simulink model "endocrino"  (R2026b)
settings: Solver=ode15s  StopTime=10  MaxStep=1E-3
libraries: slpidlib x1
settings Model: Creator=BioMath  LastModifiedBy=Emiliano
settings DataIOCC: DSMLogging=off  ReturnWorkspaceOutputs=off  SaveOutput=off  SignalLogging=off  TimeSaveName=t
settings DebuggingCC: AlgebraicLoopMsg=none  ArtificialAlgebraicLoopMsg=none  MaxConsecutiveZCsMsg=none

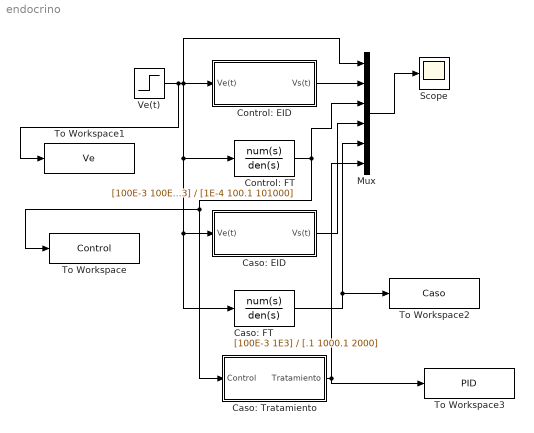
== system endocrino ==
  Caso: EID : Subsystem
  Caso: FT : TransferFcn  Numerator=[100E-3 1E3]  Denominator=[.1 1000.1 2000]
  Caso: Tratamiento : Subsystem
  Control: EID : Subsystem
  Control: FT : TransferFcn  Numerator=[100E-3 100E3]  Denominator=[1E-4 100.1 101000]
  Mux : Mux  Inputs=6
  Scope : Scope
      settings: ActiveDisplayYMinimum=0  ActiveDisplayYMaximum=1.1
  To Workspace : ToWorkspace  VariableName=Control  SampleTime=-1
  To Workspace1 : ToWorkspace  VariableName=Ve  SampleTime=-1
  To Workspace2 : ToWorkspace  VariableName=Caso  SampleTime=-1
  To Workspace3 : ToWorkspace  VariableName=PID  SampleTime=-1
  Ve(t) : Step  Time=0  SampleTime=0
  wires:
  Ve(t)/1 -> To Workspace1/1, Caso: FT/1, Caso: EID/1(Ve(t)), Control: FT/1, Control: EID/1(Ve(t)), Mux/1
  Control: EID/1(Vs(t)) -> Mux/2
  Mux/1 -> Scope/1
  Control: FT/1 -> To Workspace/1, Caso: Tratamiento/1(Control), Mux/3
  Caso: EID/1(Vs(t)) -> Mux/4
  Caso: FT/1 -> To Workspace2/1, Mux/5
  Caso: Tratamiento/1(Tratamiento) -> Mux/6, To Workspace3/1

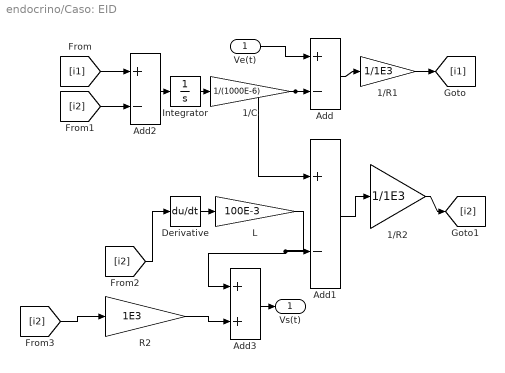
== system endocrino/Caso: EID ==
  Ve(t) : Inport
  1/C : Gain  Gain=1/(1000E-6)
  1/R1 : Gain  Gain=1/1E3
  1/R2 : Gain  Gain=1/1E3
  Add : Sum  Inputs=+-
  Add1 : Sum  Inputs=+-
  Add2 : Sum  Inputs=+-
  Add3 : Sum
  Derivative : Derivative
  Integrator : Integrator
  L : Gain  Gain=100E-3
  R2 : Gain  Gain=1E3
  Vs(t) : Outport
  wires:
  Add1/1 -> 1/R2/1
  1/R2/1 -> [i2]
  Derivative/1 -> L/1
  L/1 -> Add3/1, Add1/2
  1/R1/1 -> [i1]
  Add/1 -> 1/R1/1
  Ve(t)/1 -> Add/1
  [i2] -> Add2/2
  [i1] -> Add2/1
  Add2/1 -> Integrator/1
  Integrator/1 -> 1/C/1
  1/C/1 -> Add1/1, Add/2
  [i2] -> Derivative/1
  [i2] -> R2/1
  R2/1 -> Add3/2
  Add3/1 -> Vs(t)/1

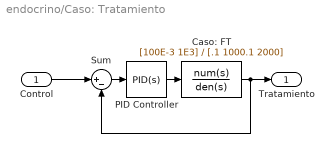
== system endocrino/Caso: Tratamiento ==
  Control : Inport
  Caso: FT : TransferFcn  Numerator=[100E-3 1E3]  Denominator=[.1 1000.1 2000]
  PID Controller : slpidlib/PID Controller  Controller=PID  Form=Parallel  TimeDomain=Continuous-time  UseExternalTs=off  SampleTime=-1  IntegratorMethod=Forward Euler  FilterMethod=Forward Euler  ControllerParametersSource=internal  P=529.0879  I=51836.0493  UseKiTs=off  D=0.17756  UseExternalDerivativeSource=off  N=2021.2211  UseFilter=on  TunerSelectOption=Transfer Function Based (PID Tuner App)  InitialConditionSource=internal  InitialConditionForIntegrator=0  InitialConditionForFilter=0  DifferentiatorICPrevScaledInput=0  ExternalReset=none  TrackingMode=off  Kt=1  LimitOutput=off  SatLimitsSource=internal  UpperSaturationLimit=inf  LowerSaturationLimit=-inf  LinearizeAsGain=on  AntiWindupMode=none  Kb=1  LimitIntegrator=off  UpperIntegratorSaturationLimit=inf  LowerIntegratorSaturationLimit=-inf  POutMin=[]  POutMax=[]  IOutMin=[]  IOutMax=[]  DOutMin=[]  DOutMax=[]  NOutMin=[]  NOutMax=[]  SumOutMin=[]  SumOutMax=[]  SaturationOutMin=[]  SaturationOutMax=[]  PParamMin=[]  PParamMax=[]  IParamMin=[]  IParamMax=[]  DParamMin=[]  DParamMax=[]  NParamMin=[]  NParamMax=[]  KbParamMin=[]  KbParamMax=[]  KtParamMin=[]  KtParamMax=[]  KbOutMin=[]  KbOutMax=[]  KtOutMin=[]  KtOutMax=[]  IntegratorOutMin=[]  IntegratorOutMax=[]  FilterOutMin=[]  FilterOutMax=[]  SumI1OutMin=[]  SumI1OutMax=[]  SumI2OutMin=[]  SumI2OutMax=[]  SumI3OutMin=[]  SumI3OutMax=[]  SumI4OutMin=[]  SumI4OutMax=[]  SumDOutMin=[]  SumDOutMax=[]  DifferentiatorOutMin=[]  DifferentiatorOutMax=[]  FilterDiffOutCoefMin=[]  FilterDiffOutCoefMax=[]  ReciprocalOutMin=[]  ReciprocalOutMax=[]  SumDenOutMin=[]  SumDenOutMax=[]  SumNumOutMin=[]  SumNumOutMax=[]  DivideOutMin=[]  DivideOutMax=[]  UdiffTsProdOutMin=[]  UdiffTsProdOutMax=[]  NTsProdOutMin=[]  NTsProdOutMax=[]  UintegralTsProdOutMin=[]  UintegralTsProdOutMax=[]  UngainTsProdOutMin=[]  UngainTsProdOutMax=[]  ClampingZeroOutDataTypeStr=Inherit: Inherit via back propagation  ClampingZeroOutMin=[]  ClampingZeroOutMax=[]  FilterDenConstantOutDataTypeStr=Inherit: Inherit via back propagation  FilterDenConstantOutMin=[]  FilterDenConstantOutMax=[]  PCopyOutDataTypeStr=Inherit: Inherit via back propagation  PCopyOutMin=[]  PCopyOutMax=[]  NCopyOutDataTypeStr=Inherit: Inherit via back propagation  NCopyOutMin=[]  NCopyOutMax=[]  IntegratorContinuousStateAttributes=''  IntegratorStateMustResolveToSignalObject=off  IntegratorRTWStateStorageClass=Auto  FilterContinuousStateAttributes=''  FilterStateMustResolveToSignalObject=off  FilterRTWStateStorageClass=Auto  ParallelPVariant=InternalParameters  IdealPVariant=Disabled  IVariant=InternalParameters  DVariant=InternalParameters  IntegratorVariant=Continuous  SatVariant=Disabled  AWVariant=Passthrough  PCopyVariant=Disabled  TRVariant=Disabled  FdbkBlocksVariant=Forward  IdealPFdbkVariant=Disabled  SatFdbkVariant=Disabled  DerivativeFilterVariant=ContFilter  NVariant=InternalParameters  NCopyVariant=Disabled  FilterICVariant=InternalICsFilter  IntegratorICVariant=InternalICs  ExternalResetVariant=Disabled  TRSumVariant=Passthrough  SumFdbkVariant=Disabled  SumVariant=Sum_PID  TsampFilterVariant=InternalTs  TsampNgainVariant=Passthrough  TsampIntegralVariant=Disabled_SignalSpec  ExternalSaturationOutDataTypeStr=Inherit: Same as second input  DerivativeSourceVariant=ErrorSignal  PreIntVariant=InternalPreInt
  Sum : Sum  Inputs=|+-
  Tratamiento : Outport
  wires:
  Control/1 -> Sum/1
  Caso: FT/1 -> Sum/2, Tratamiento/1
  Sum/1 -> PID Controller/1
  PID Controller/1 -> Caso: FT/1

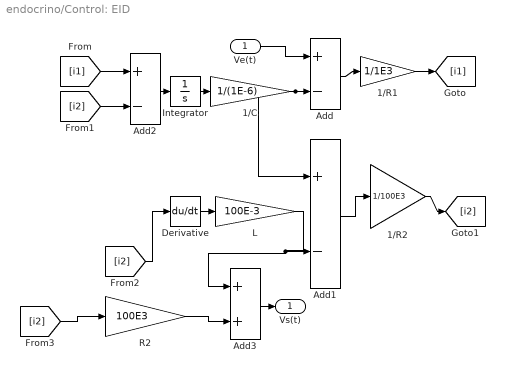
== system endocrino/Control: EID ==
  Ve(t) : Inport
  1/C : Gain  Gain=1/(1E-6)
  1/R1 : Gain  Gain=1/1E3
  1/R2 : Gain  Gain=1/100E3
  Add : Sum  Inputs=+-
  Add1 : Sum  Inputs=+-
  Add2 : Sum  Inputs=+-
  Add3 : Sum
  Derivative : Derivative
  Integrator : Integrator
  L : Gain  Gain=100E-3
  R2 : Gain  Gain=100E3
  Vs(t) : Outport
  wires:
  Add1/1 -> 1/R2/1
  1/R2/1 -> [i2]
  Derivative/1 -> L/1
  L/1 -> Add3/1, Add1/2
  1/R1/1 -> [i1]
  Add/1 -> 1/R1/1
  Ve(t)/1 -> Add/1
  [i2] -> Add2/2
  [i1] -> Add2/1
  Add2/1 -> Integrator/1
  Integrator/1 -> 1/C/1
  1/C/1 -> Add1/1, Add/2
  [i2] -> Derivative/1
  [i2] -> R2/1
  R2/1 -> Add3/2
  Add3/1 -> Vs(t)/1
